simulink model "chaine_qpsk"  (R2026b)
settings: Solver=FixedStepDiscrete  StopTime=1000  FixedStep=1
values from neighbouring files (symbols this model uses):
  graine = round(P.graine)    [Parametres.m]    (also in Partie2.m = P.graine; parametres_perso.m = mod(sum(c .* (1:numel(c)) * 31) + 7 * numel(c), 2^31 - 1))
  sig2 = 0.25/EbN0    [test_qpsk.m]    (also in test_qpsk_cod.m = (7/16)/EbN0)
libraries: simulink x1
settings Model: Creator=INS NAWEL  LastModifiedBy=INS NAWEL

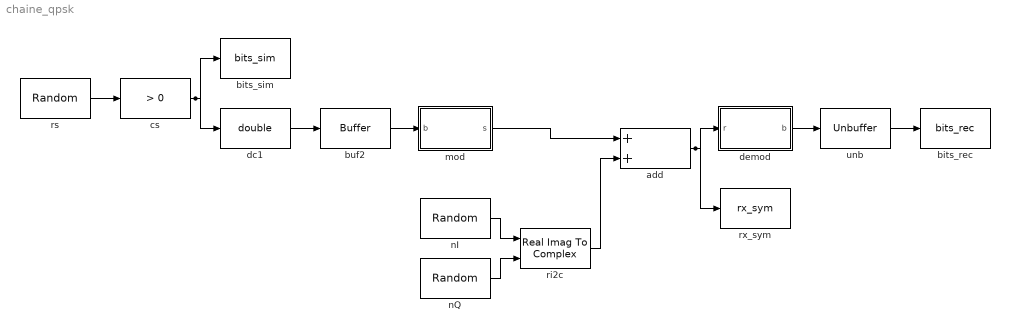
== system chaine_qpsk ==
  add : Sum
  bits_rec : ToWorkspace  VariableName=bits_rec  SampleTime=1
  bits_sim : ToWorkspace  VariableName=bits_sim  SampleTime=1
  buf2 : Buffer  N=2
  cs : simulink/Logic and Bit Operations/Compare To Constant  relop=>  const=0  OutDataTypeStr=boolean
  dc1 : DataTypeConversion  OutDataTypeStr=double  SaturateOnIntegerOverflow=off  RndMeth=Floor
  demod : MATLAB Function  TreatAsAtomicUnit=on
  mod : MATLAB Function  TreatAsAtomicUnit=on
  nI : RandomNumber  Variance=sig2  Seed=graine+2  SampleTime=2
  nQ : RandomNumber  Variance=sig2  Seed=graine+3  SampleTime=2
  ri2c : RealImagToComplex
  rs : RandomNumber  Seed=graine+1  SampleTime=1
  rx_sym : ToWorkspace  VariableName=rx_sym  SampleTime=2
  unb : Unbuffer
  wires:
  rs/1 -> cs/1
  cs/1 -> bits_sim/1, dc1/1
  dc1/1 -> buf2/1
  buf2/1 -> mod/1(b)
  mod/1(s) -> add/1
  nI/1 -> ri2c/1
  nQ/1 -> ri2c/2
  ri2c/1 -> add/2
  add/1 -> rx_sym/1, demod/1(r)
  demod/1(b) -> unb/1
  unb/1 -> bits_rec/1

== matlab function chaine_qpsk/mod ==
  data: b input; s output
function s = qpsk_mod(b)
%#codegen
b = double(b(:));
k = 1 + 2*(2*b(1) + b(2));
s = exp(1j*pi/4*k);
end

== matlab function chaine_qpsk/demod ==
  data: r input; b output
function b = qpsk_demod(r)
%#codegen
bi = double(real(r) < 0);
bq = double(imag(r) < 0);
b = [bq; mod(bi + bq, 2)];
end
